simulink model "rfdctxrx"  (R2025a)
settings: Solver=VariableStepAuto  StartTime=0.0  StopTime=10.0  RelTol=1e-3
libraries: hdlBasic x265, casper_library_misc x2, xps_library x1, vmcUtilities x1
(part 5 of 7)

== system rfdctxrx/tx_enable ==
  sim_1 : Inport
  convert1_1 : DataTypeConversion  OutDataTypeStr=fixdt('ufix1_En0')  SaturateOnIntegerOverflow=off  RndMeth=Floor  LockScale=on
  convert2_1 : DataTypeConversion  OutDataTypeStr=fixdt('ufix1_En0')  ConvertRealWorld=Stored Integer (SI)  SaturateOnIntegerOverflow=off  RndMeth=Floor  LockScale=on
  gain_1 : Gain  OutDataTypeStr=fixdt('ufix32_En0')
  io_delay : hdlBasic/Delay  rst=off  en=off  latency=0  reg_retiming=on  XmcBlockStatus=0  maskContainerNames=group1  block_type=delay  block_config=sysgen:Delay_config
  rfdctxrx_tx_enable_user_data_out : hdlBasic/Gateway In  gui_display_data_type=Fixed-point  arith_type=Unsigned  n_bits=32  bin_pt=0  preci_type=Single  exp_width=8  frac_width=24  rows=1  columns=1  quantization="Round  (unbiased: +/- Inf)"  overflow=Saturate  period=1  UseAsADC=off  ADCChannel='1'  interface=None  automatic_assignment=on  address_offset=hex2dec('00')  intf_name=''  intf_description=''  default_value=0  timing_constraint=None  locs_specified=off  LOCs={}  io_standard={}  inherit_from_input=off  hdl_port=on  XmcBlockStatus=0  maskContainerNames=group4  block_type=gatewayin  block_config=sysgen:gateway_in_config  block_width_w=590  block_height_w=620  block_width=640  block_height=850
  slice_reg : hdlBasic/Slice  nbits=1  boolean_output=on  mode=Lower Bit Location + Width  bit1=0  base1=MSB of Input  bit0=0  base0=LSB of Input  XmcBlockStatus=0  maskContainerNames=group1  block_type=slice  block_config=sysgen:Slice_config
  in_reg : Outport
  wires:
  rfdctxrx_tx_enable_user_data_out/1 -> io_delay/1
  sim_1/1 -> convert1_1/1
  convert1_1/1 -> convert2_1/1
  convert2_1/1 -> gain_1/1
  gain_1/1 -> rfdctxrx_tx_enable_user_data_out/1
  io_delay/1 -> slice_reg/1
  slice_reg/1 -> in_reg/1

== system rfdctxrx/tx_len ==
  out_reg : Inport
  assert_reg : hdlBasic/Assert  assert_type=on  type_source=Explicitly  gui_display_data_type=Fixed-point  arith_type=Unsigned  n_bits=13  bin_pt=0  preci_type=Single  exp_width=8  frac_width=24  assert_rate=off  rate_source=Explicitly  period=1  output_port=on  XmcBlockStatus=0  maskContainerNames=group1  block_type=assert  block_config=sysgen:assert_config  block_width=609  block_height=900
  cast_gw : hdlBasic/Convert  gui_display_data_type=Fixed-point  arith_type=Unsigned  n_bits=32  bin_pt=0  float_type=Single  exp_bits=8  fraction_bits=24  quantization=Truncate  overflow=Wrap  en=off  latency=1  pipeline=off  XmcBlockStatus=0  maskContainerNames=group2  block_type=convert  block_config=sysgen:Convert_config  block_width=595  block_height=885
  io_delay : hdlBasic/Delay  rst=off  en=off  latency=0  reg_retiming=on  XmcBlockStatus=0  maskContainerNames=group1  block_type=delay  block_config=sysgen:Delay_config
  reint1 : hdlBasic/Reinterpret  force_arith_type=on  arith_type=Unsigned  force_bin_pt=on  bin_pt=0  XmcBlockStatus=0  maskContainerNames=group1  block_type=reinterpret  block_config=sysgen:Reinterpret_config
  rfdctxrx_tx_len_user_data_in : hdlBasic/Gateway Out  inherit_from_input=off  bool_to_boolean=off  hdl_port=on  rows=1  columns=1  UseAsDAC=off  DACChannel='1'  interface=None  automatic_assignment=on  address_offset=hex2dec('00')  intf_name=''  intf_description=''  timing_constraint=None  locs_specified=off  LOCs={}  io_standard={}  XmcBlockStatus=0  maskContainerNames=group4  block_type=gatewayout  block_config=sysgen:gateway_out_config  block_width_w=590  block_height_w=620  block_width=620  block_height=750
  sim_out : Terminator
  sim_out_reg_gw : hdlBasic/Gateway Out  inherit_from_input=off  bool_to_boolean=off  hdl_port=off  rows=1  columns=1  UseAsDAC=off  DACChannel='1'  interface=None  automatic_assignment=on  address_offset=hex2dec('00')  intf_name=''  intf_description=''  timing_constraint=None  locs_specified=off  LOCs={}  io_standard={}  XmcBlockStatus=0  maskContainerNames=group4  block_type=gatewayout  block_config=sysgen:gateway_out_config  block_width_w=590  block_height_w=620  block_width=620  block_height=750
  sim_out_reg_sim_delay : hdlBasic/Delay  rst=off  en=off  latency=1  reg_retiming=on  XmcBlockStatus=0  maskContainerNames=group1  block_type=delay  block_config=sysgen:Delay_config
  sim_out_reg : Outport  VectorParamsAs1DForOutWhenUnconnected=off
  wires:
  sim_out_reg_sim_delay/1 -> sim_out_reg_gw/1
  sim_out_reg_gw/1 -> sim_out_reg/1
  io_delay/1 -> cast_gw/1
  cast_gw/1 -> rfdctxrx_tx_len_user_data_in/1
  rfdctxrx_tx_len_user_data_in/1 -> sim_out/1
  out_reg/1 -> sim_out_reg_sim_delay/1, assert_reg/1
  assert_reg/1 -> reint1/1
  reint1/1 -> io_delay/1

== system rfdctxrx/bitfield_snapshot/buscreate ==
  in1 : Inport
  in2 : Inport  Port=2
  concatenate : hdlBasic/Concat  num_inputs=2  XmcBlockStatus=1  maskContainerNames=group1  block_type=concat  block_config=sysgen:Concat_config
  reinterpret1 : hdlBasic/Reinterpret  force_arith_type=on  arith_type=Unsigned  force_bin_pt=on  bin_pt=0  XmcBlockStatus=1  maskContainerNames=group1  block_type=reinterpret  block_config=sysgen:Reinterpret_config
  reinterpret2 : hdlBasic/Reinterpret  force_arith_type=on  arith_type=Unsigned  force_bin_pt=on  bin_pt=0  XmcBlockStatus=1  maskContainerNames=group1  block_type=reinterpret  block_config=sysgen:Reinterpret_config
  bus_out : Outport  VectorParamsAs1DForOutWhenUnconnected=off
  wires:
  concatenate/1 -> bus_out/1
  in1/1 -> reinterpret1/1
  reinterpret1/1 -> concatenate/1
  in2/1 -> reinterpret2/1
  reinterpret2/1 -> concatenate/2

== system rfdctxrx/bitfield_snapshot/io_delay ==
  d : Inport
  Register0 : hdlBasic/Register  init=0  rst=off  en=off  XmcBlockStatus=1  maskContainerNames=tabcontainer1  block_type=register  block_config=sysgen:Register_config
  Register1 : hdlBasic/Register  init=0  rst=off  en=off  XmcBlockStatus=1  maskContainerNames=tabcontainer1  block_type=register  block_config=sysgen:Register_config
  q : Outport  VectorParamsAs1DForOutWhenUnconnected=off
  wires:
  Register1/1 -> q/1
  d/1 -> Register0/1
  Register0/1 -> Register1/1

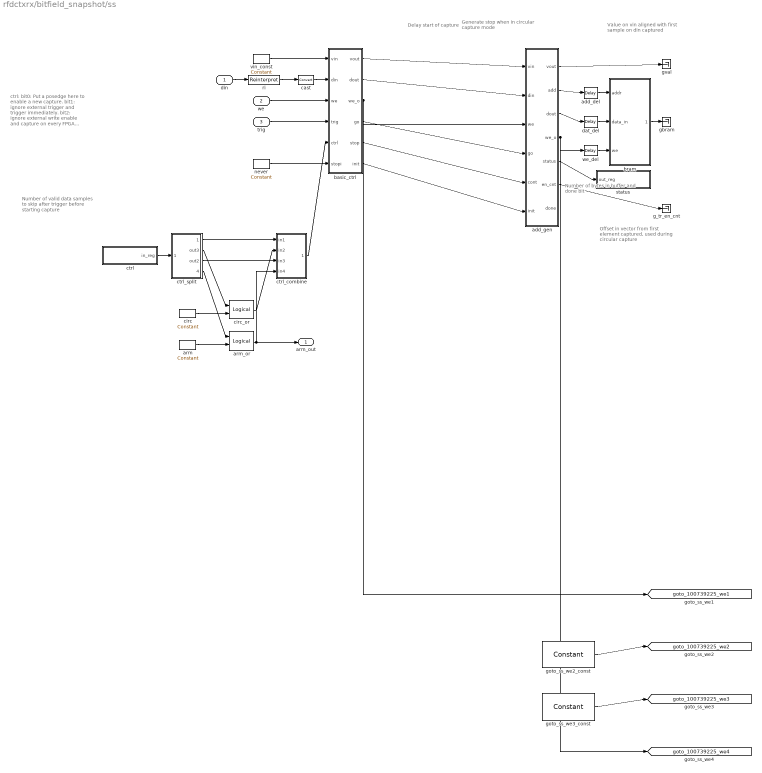
== system rfdctxrx/bitfield_snapshot/ss ==
  note: Generate stop
      | when in circular
      | capture mode
  note: Delay start
      | of capture
  note: ctrl:
      | bit0: Put a posedge here
      |         to enable a new capture.
      | bit1: ignore external trigger
      |         and trigger immediately.
      | bit2: ignore external write
      |         enable and capture on
      |         every FPGA clock.
      | bit3: continuously capture
      |         data until we get an
      |         external stop command.
  note: Offset in vector
      | from first element
      | captured, used
      | during circular capture
  note: Number of
      | bytes in
      | buffer and
      | done bit
  note: Number of valid
      | data samples to
      | skip after trigger
      | before starting
      | capture
  note: Value on vin
      | aligned with
      | first sample on
      | din captured
  din : Inport
  we : Inport  Port=2
  trig : Inport  Port=3
  add_del : hdlBasic/Delay  rst=off  en=off  latency=1  reg_retiming=off  XmcBlockStatus=1  maskContainerNames=group1  block_type=delay  block_config=sysgen:Delay_config
  add_gen : Subsystem  AncestorBlock=casper_library_scopes/snapshot/add_gen  mask{counter_size=14+4+1, increment=16, nsamples=14, burst_size=0, use_dsp48=on}
      mask prompts: counter_size "Address counter size (2^?)"; increment "Address counter increment"; nsamples "Number of samples (2^?)"; burst_size "Burst size (2^?)"; use_dsp48 "dsp48 counter/s"
      mask init:
      | set_param(gcb,'LinkStatus','inactive');
      | if strcmp(use_dsp48,'on'),
      |     set_param([gcb,'/add_gen'],'implementation','DSP48');
      | else
      |     set_param([gcb,'/add_gen'],'implementation','Fabric');
      | end
  arm : hdlBasic/Constant  const=0  gui_display_data_type=Boolean  arith_type=Boolean  n_bits=16  bin_pt=14  preci_type=Single  exp_width=8  frac_width=24  explicit_period=on  period=1  XmcBlockStatus=1  maskContainerNames=tabcontainer1  block_type=constant  block_config=sysgen:Constant_config
  arm_or : hdlBasic/Logical  logical_function=OR  inputs=2  en=off  latency=0  precision=Full  arith_type=Unsigned  n_bits=16  bin_pt=0  align_bp=on  overflow=[]  quantization=[]  XmcBlockStatus=1  maskContainerNames=tabcontainer1  block_type=logical  block_config=sysgen:Logical_config
  basic_ctrl : Subsystem  AncestorBlock=casper_library_scopes/snapshot/basic_ctrl  mask{dram=off, data_width=128}
      mask prompts: data_width "data width"
      mask init:
      | set_param(gcb,'LinkStatus','inactive');
      | set_param([gcb,'/dram_munge'], 'dram', dram);
  bram : Subsystem  Tag=xps:bram  AncestorBlock=xps_library/Memory/shared_bram  mask{arith_type=Unsigned, addr_width=14, data_width=128, reg_prim_output=off, reg_core_output=off, optimization=Minimum_Area, data_bin_pt=0, init_vals=[0:2^14-1], sample_rate=1}
      mask prompts: arith_type "Output Data Type"; addr_width "Address width"; data_width "Data Width"; reg_prim_output "Register Primitive Output"; reg_core_output "Register Core Output"; data_bin_pt "Data Binary Point"; init_vals "Initial values (simulation only)"; sample_rate "Sample rate"
      mask init:
      | shared_bram_mask;
      mask TypeOptions arith_type: Unsigned | Signed  (2's comp)
      mask TypeOptions data_width: 8 | 16 | 32 | 64 | 128
      mask TypeOptions optimization: Minimum_Area | Low_Power
  cast : hdlBasic/Convert  gui_display_data_type=Fixed-point  arith_type=Unsigned  n_bits=128  bin_pt=0  float_type=Single  exp_bits=8  fraction_bits=24  quantization=Truncate  overflow=Wrap  en=off  latency=0  pipeline=off  XmcBlockStatus=1  maskContainerNames=group2  block_type=convert  block_config=sysgen:Convert_config  block_width=595  block_height=885
  circ : hdlBasic/Constant  const=0  gui_display_data_type=Boolean  arith_type=Boolean  n_bits=16  bin_pt=14  preci_type=Single  exp_width=8  frac_width=24  explicit_period=on  period=1  XmcBlockStatus=1  maskContainerNames=tabcontainer1  block_type=constant  block_config=sysgen:Constant_config
  circ_or : hdlBasic/Logical  logical_function=OR  inputs=2  en=off  latency=0  precision=Full  arith_type=Unsigned  n_bits=16  bin_pt=0  align_bp=on  overflow=[]  quantization=[]  XmcBlockStatus=1  maskContainerNames=tabcontainer1  block_type=logical  block_config=sysgen:Logical_config
  ctrl : Subsystem  Tag=xps:sw_reg  AncestorBlock=xps_library/Memory/software_register  mask(swreg){io_dir=From Processor, io_delay=0, init_val=0, sample_period=1, names=reg, bitwidths=32, bin_pts=0, arith_types=0, sim_port=off, show_format=on}
      mask prompts: io_dir "I/O direction"; io_delay "I/O delay"; init_val "Initial Value"; sample_period "Sample period"; names "Bitfield names [msb...lsb]"; bitwidths "Bitfield widths"; bin_pts "Bitfield binary pts"; arith_types "Bitfield types, ufix=0, fix=1, bool=2"; sim_port "Provide sim input/output?"; show_format "Print format string?"
      mask help: A 32-bit software-accessible register. Can be divided into bitfields of varying widths and types using the fields in the block mask.
      mask init:
      | swreg_init(gcb)
      settings: AttributesFormatString=1input:uf32.0 = 32 bits
      mask TypeOptions io_dir: To Processor | From Processor
      mask Callback io_dir:
      | mask_enables = get_param(gcb, 'MaskEnables');
      | mask_names = get_param(gcb, 'MaskNames');
      | if strcmp(get_param(gcb, 'io_dir'), 'To Processor'),
      |     mask_enables{ismember(mask_names, 'sample_period')} = 'off';
      | else
      |     mask_enables{ismember(mask_names, 'sample_period')} = 'on';
      | end
      | set_param(gcb, 'MaskEnables', mask_enables);
      mask DialogControl ParameterTabVar0 Prompt: Setup
  ctrl_combine : Subsystem  AncestorBlock=casper_library_flow_control/bus_create  mask(bus_create){inputNum=4}
      mask prompts: inputNum "Number of inputs:"
      mask init:
      | bus_create_init(gcb,...
      |     'inputNum', inputNum);
  ctrl_split : Subsystem  AncestorBlock=casper_library_flow_control/bus_expand  mask(bus_expand){mode=divisions of arbitrary size, outputNum=1, outputWidth=[28 1 2 1], outputBinaryPt=0, outputArithmeticType=[0 2 0 2], show_format=on, outputToWorkspace=off, variablePrefix=out, outputToModelAsWell=on}
      mask prompts: outputNum "Number of outputs:"; outputWidth "Output width [msb ... lsb]:"; outputBinaryPt "Output binary point position [msb ... lsb]:"; outputArithmeticType "Output arithmetic type (ufix=0, fix=1, bool=2) [msb ... lsb]:"; show_format "Print format string?"; outputToWorkspace "Output to workspace?"; variablePrefix "Variable name prefix:"; outputToModelAsWell "Output to model as well?"
      mask help:
      | Expands a 'bus' made using a bus_create or Xilinx
      | concat block.
      | The input will be divided into the specified number
      | of outputs with the specified arithmetic types.
      | Divisions are made from most significant bit.
      mask init: same as rfdctxrx/munge/split
      settings: AttributesFormatString=4 outputs: uf28.0,b,uf2.0,b,
      mask TypeOptions mode: divisions of equal size | divisions of arbitrary size
      mask Callback mode: bus_expand_callback();
      mask Callback outputWidth: bus_expand_callback();
      mask Callback outputToWorkspace: bus_expand_callback();
  dat_del : hdlBasic/Delay  rst=off  en=off  latency=1  reg_retiming=off  XmcBlockStatus=1  maskContainerNames=group1  block_type=delay  block_config=sysgen:Delay_config
  g_tr_en_cnt : Terminator
  gbram : Terminator
  goto_ss_we2_const : hdlBasic/Constant  const=0  gui_display_data_type=Boolean  arith_type=Boolean  n_bits=16  bin_pt=14  preci_type=Single  exp_width=8  frac_width=24  explicit_period=on  period=1  XmcBlockStatus=1  maskContainerNames=tabcontainer1  block_type=constant  block_config=sysgen:Constant_config
  goto_ss_we3_const : hdlBasic/Constant  const=0  gui_display_data_type=Boolean  arith_type=Boolean  n_bits=16  bin_pt=14  preci_type=Single  exp_width=8  frac_width=24  explicit_period=on  period=1  XmcBlockStatus=1  maskContainerNames=tabcontainer1  block_type=constant  block_config=sysgen:Constant_config
  gval : Terminator
  never : hdlBasic/Constant  const=0  gui_display_data_type=Boolean  arith_type=Boolean  n_bits=16  bin_pt=14  preci_type=Single  exp_width=8  frac_width=24  explicit_period=on  period=1  XmcBlockStatus=1  maskContainerNames=tabcontainer1  block_type=constant  block_config=sysgen:Constant_config
  ri : hdlBasic/Reinterpret  force_arith_type=on  arith_type=Unsigned  force_bin_pt=on  bin_pt=0  XmcBlockStatus=1  maskContainerNames=group1  block_type=reinterpret  block_config=sysgen:Reinterpret_config
  status : Subsystem  Tag=xps:sw_reg  AncestorBlock=xps_library/Memory/software_register  mask(swreg){io_dir=To Processor, io_delay=0, init_val=0, sample_period=1, names=reg, bitwidths=32, bin_pts=0, arith_types=0, sim_port=off, show_format=on}
      mask prompts: io_dir "I/O direction"; io_delay "I/O delay"; init_val "Initial Value"; sample_period "Sample period"; names "Bitfield names [msb...lsb]"; bitwidths "Bitfield widths"; bin_pts "Bitfield binary pts"; arith_types "Bitfield types, ufix=0, fix=1, bool=2"; sim_port "Provide sim input/output?"; show_format "Print format string?"
      mask help: A 32-bit software-accessible register. Can be divided into bitfields of varying widths and types using the fields in the block mask.
      mask init:
      | swreg_init(gcb)
      settings: AttributesFormatString=1output:uf32.0 = 32 bits
      mask TypeOptions io_dir: To Processor | From Processor
      mask Callback io_dir:
      | mask_enables = get_param(gcb, 'MaskEnables');
      | mask_names = get_param(gcb, 'MaskNames');
      | if strcmp(get_param(gcb, 'io_dir'), 'To Processor'),
      |     mask_enables{ismember(mask_names, 'sample_period')} = 'off';
      | else
      |     mask_enables{ismember(mask_names, 'sample_period')} = 'on';
      | end
      | set_param(gcb, 'MaskEnables', mask_enables);
      mask DialogControl ParameterTabVar0 Prompt: Setup
  vin_const : hdlBasic/Constant  const=0  gui_display_data_type=Boolean  arith_type=Boolean  n_bits=16  bin_pt=14  preci_type=Single  exp_width=8  frac_width=24  explicit_period=on  period=1  XmcBlockStatus=1  maskContainerNames=tabcontainer1  block_type=constant  block_config=sysgen:Constant_config
  we_del : hdlBasic/Delay  rst=off  en=off  latency=1  reg_retiming=off  XmcBlockStatus=1  maskContainerNames=group1  block_type=delay  block_config=sysgen:Delay_config
  arm_out : Outport  VectorParamsAs1DForOutWhenUnconnected=off
  tag scope: goto_100739225_we1=global, goto_100739225_we2=global, goto_100739225_we3=global, goto_100739225_we4=global
  wires:
  din/1 -> ri/1
  ri/1 -> cast/1
  cast/1 -> basic_ctrl/2(din)
  we/1 -> basic_ctrl/3(we)
  trig/1 -> basic_ctrl/4(trig)
  ctrl_combine/1(bus_out) -> basic_ctrl/5(ctrl)
  never/1 -> basic_ctrl/6(stopi)
  arm/1 -> arm_or/2
  arm_or/1 -> arm_out/1, ctrl_combine/4(in4)
  circ/1 -> circ_or/2
  ctrl/1(in_reg) -> ctrl_split/1(bus_in)
  ctrl_split/1(msb_out4) -> ctrl_combine/1(in1)
  ctrl_split/2(out3) -> circ_or/1
  ctrl_split/3(out2) -> ctrl_combine/3(in3)
  ctrl_split/4(lsb_out1) -> arm_or/1
  circ_or/1 -> ctrl_combine/2(in2)
  basic_ctrl/1(vout) -> add_gen/1(vin)
  basic_ctrl/2(dout) -> add_gen/2(din)
  basic_ctrl/3(we_o) -> add_gen/3(we), [goto_100739225_we1]
  basic_ctrl/4(go) -> add_gen/4(go)
  basic_ctrl/5(stop) -> add_gen/5(cont)
  basic_ctrl/6(init) -> add_gen/6(init)
  add_gen/5(status) -> status/1(out_reg)
  vin_const/1 -> basic_ctrl/1(vin)
  add_gen/1(vout) -> gval/1
  add_gen/6(en_cnt) -> g_tr_en_cnt/1
  add_gen/2(add) -> add_del/1
  add_gen/3(dout) -> dat_del/1
  add_gen/4(we_o) -> we_del/1, [goto_100739225_we4]
  add_del/1 -> bram/1(addr)
  dat_del/1 -> bram/2(data_in)
  we_del/1 -> bram/3(we)
  bram/1(data_out) -> gbram/1
  goto_ss_we2_const/1 -> [goto_100739225_we2]
  goto_ss_we3_const/1 -> [goto_100739225_we3]

== system rfdctxrx/bitfield_snapshot/trig_delay ==
  d : Inport
  Register0 : hdlBasic/Register  init=0  rst=off  en=off  XmcBlockStatus=1  maskContainerNames=tabcontainer1  block_type=register  block_config=sysgen:Register_config
  Register1 : hdlBasic/Register  init=0  rst=off  en=off  XmcBlockStatus=1  maskContainerNames=tabcontainer1  block_type=register  block_config=sysgen:Register_config
  q : Outport  VectorParamsAs1DForOutWhenUnconnected=off
  wires:
  Register1/1 -> q/1
  d/1 -> Register0/1
  Register0/1 -> Register1/1

== system rfdctxrx/bitfield_snapshot/we_delay ==
  d : Inport
  Register0 : hdlBasic/Register  init=0  rst=off  en=off  XmcBlockStatus=1  maskContainerNames=tabcontainer1  block_type=register  block_config=sysgen:Register_config
  Register1 : hdlBasic/Register  init=0  rst=off  en=off  XmcBlockStatus=1  maskContainerNames=tabcontainer1  block_type=register  block_config=sysgen:Register_config
  q : Outport  VectorParamsAs1DForOutWhenUnconnected=off
  wires:
  Register1/1 -> q/1
  d/1 -> Register0/1
  Register0/1 -> Register1/1

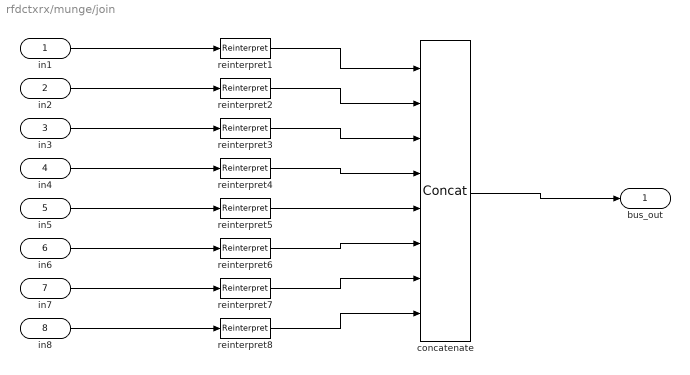
== system rfdctxrx/munge/join ==
  in1 : Inport
  in2 : Inport  Port=2
  in3 : Inport  Port=3
  in4 : Inport  Port=4
  in5 : Inport  Port=5
  in6 : Inport  Port=6
  in7 : Inport  Port=7
  in8 : Inport  Port=8
  concatenate : hdlBasic/Concat  num_inputs=8  XmcBlockStatus=1  maskContainerNames=group1  block_type=concat  block_config=sysgen:Concat_config
  reinterpret{1..8} (8 alike) : hdlBasic/Reinterpret  force_arith_type=on  arith_type=Unsigned  force_bin_pt=on  bin_pt=0  XmcBlockStatus=1  maskContainerNames=group1  block_type=reinterpret  block_config=sysgen:Reinterpret_config
  bus_out : Outport  VectorParamsAs1DForOutWhenUnconnected=off
  wires:
  concatenate/1 -> bus_out/1
  in1/1 -> reinterpret1/1
  reinterpret1/1 -> concatenate/1
  in2/1 -> reinterpret2/1
  reinterpret2/1 -> concatenate/2
  in3/1 -> reinterpret3/1
  reinterpret3/1 -> concatenate/3
  in4/1 -> reinterpret4/1
  reinterpret4/1 -> concatenate/4
  in5/1 -> reinterpret5/1
  reinterpret5/1 -> concatenate/5
  in6/1 -> reinterpret6/1
  reinterpret6/1 -> concatenate/6
  in7/1 -> reinterpret7/1
  reinterpret7/1 -> concatenate/7
  in8/1 -> reinterpret8/1
  reinterpret8/1 -> concatenate/8

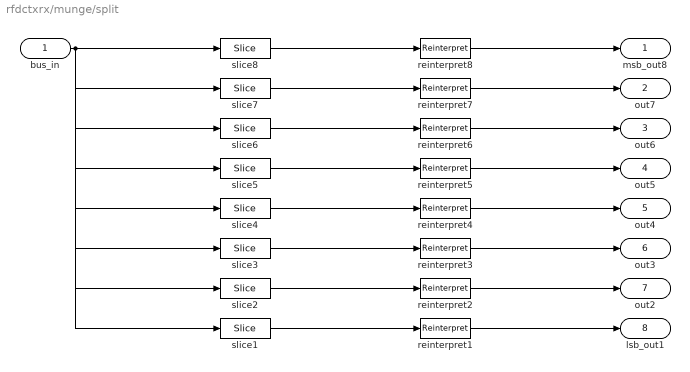
== system rfdctxrx/munge/split ==
  bus_in : Inport
  reinterpret{1..8} (8 alike) : hdlBasic/Reinterpret  force_arith_type=on  arith_type=Unsigned  force_bin_pt=on  bin_pt=0  XmcBlockStatus=1  maskContainerNames=group1  block_type=reinterpret  block_config=sysgen:Reinterpret_config
  slice1 : hdlBasic/Slice  nbits=16  boolean_output=off  mode=Upper Bit Location + Width  bit1=-112  base1=MSB of Input  bit0=0  base0=LSB of Input  XmcBlockStatus=1  maskContainerNames=group1  block_type=slice  block_config=sysgen:Slice_config
  slice2 : hdlBasic/Slice  nbits=16  boolean_output=off  mode=Upper Bit Location + Width  bit1=-96  base1=MSB of Input  bit0=0  base0=LSB of Input  XmcBlockStatus=1  maskContainerNames=group1  block_type=slice  block_config=sysgen:Slice_config
  slice3 : hdlBasic/Slice  nbits=16  boolean_output=off  mode=Upper Bit Location + Width  bit1=-80  base1=MSB of Input  bit0=0  base0=LSB of Input  XmcBlockStatus=1  maskContainerNames=group1  block_type=slice  block_config=sysgen:Slice_config
  slice4 : hdlBasic/Slice  nbits=16  boolean_output=off  mode=Upper Bit Location + Width  bit1=-64  base1=MSB of Input  bit0=0  base0=LSB of Input  XmcBlockStatus=1  maskContainerNames=group1  block_type=slice  block_config=sysgen:Slice_config
  slice5 : hdlBasic/Slice  nbits=16  boolean_output=off  mode=Upper Bit Location + Width  bit1=-48  base1=MSB of Input  bit0=0  base0=LSB of Input  XmcBlockStatus=1  maskContainerNames=group1  block_type=slice  block_config=sysgen:Slice_config
  slice6 : hdlBasic/Slice  nbits=16  boolean_output=off  mode=Upper Bit Location + Width  bit1=-32  base1=MSB of Input  bit0=0  base0=LSB of Input  XmcBlockStatus=1  maskContainerNames=group1  block_type=slice  block_config=sysgen:Slice_config
  slice7 : hdlBasic/Slice  nbits=16  boolean_output=off  mode=Upper Bit Location + Width  bit1=-16  base1=MSB of Input  bit0=0  base0=LSB of Input  XmcBlockStatus=1  maskContainerNames=group1  block_type=slice  block_config=sysgen:Slice_config
  slice8 : hdlBasic/Slice  nbits=16  boolean_output=off  mode=Upper Bit Location + Width  bit1=0  base1=MSB of Input  bit0=0  base0=LSB of Input  XmcBlockStatus=1  maskContainerNames=group1  block_type=slice  block_config=sysgen:Slice_config
  msb_out8 : Outport
  out7 : Outport  Port=2
  out6 : Outport  Port=3
  out5 : Outport  Port=4
  out4 : Outport  Port=5
  out3 : Outport  Port=6
  out2 : Outport  Port=7
  lsb_out1 : Outport  Port=8  VectorParamsAs1DForOutWhenUnconnected=off
  wires:
  bus_in/1 -> slice8/1, slice7/1, slice6/1, slice5/1, slice4/1, slice3/1, slice2/1, slice1/1
  slice8/1 -> reinterpret8/1
  reinterpret8/1 -> msb_out8/1
  slice7/1 -> reinterpret7/1
  reinterpret7/1 -> out7/1
  slice6/1 -> reinterpret6/1
  reinterpret6/1 -> out6/1
  slice5/1 -> reinterpret5/1
  reinterpret5/1 -> out5/1
  slice4/1 -> reinterpret4/1
  reinterpret4/1 -> out4/1
  slice3/1 -> reinterpret3/1
  reinterpret3/1 -> out3/1
  slice2/1 -> reinterpret2/1
  reinterpret2/1 -> out2/1
  slice1/1 -> reinterpret1/1
  reinterpret1/1 -> lsb_out1/1

== system rfdctxrx/tx_bram/calc_add ==
  note: Use behavioural HDL
      | so that gets optimised
      | to minimum logic
  note: If reading/writing words
      | smaller than 32 bits,
      | change address so
      | that addressing is
      | big endian instead of
      | little, otherwise
      | pass through
  in : Inport
  add_sub : hdlBasic/AddSub  mode=Subtraction  use_carryin=off  use_carryout=off  en=off  latency=0  precision=User Defined  arith_type=Unsigned  n_bits=max(1, log2(32/data_width))  bin_pt=0  quantization=Truncate  overflow=Wrap  use_behavioral_HDL=on  hw_selection=Fabric  pipelined=off  XmcBlockStatus=1  maskContainerNames=tabcontainer1  block_type=addsub  block_config=sysgen:Addsub_config
  concat : hdlBasic/Concat  num_inputs=2  XmcBlockStatus=1  maskContainerNames=group1  block_type=concat  block_config=sysgen:Concat_config
  const : hdlBasic/Constant  const=max(0, 32/data_width-1)  gui_display_data_type=Fixed-point  arith_type=Unsigned  n_bits=max(1, log2(32/data_width))  bin_pt=0  preci_type=Single  exp_width=8  frac_width=24  explicit_period=on  period=sample_rate  XmcBlockStatus=1  maskContainerNames=tabcontainer1  block_type=constant  block_config=sysgen:Constant_config
  convert_addr : hdlBasic/Convert  gui_display_data_type=Fixed-point  arith_type=Unsigned  n_bits=addr_width  bin_pt=0  float_type=Single  exp_bits=8  fraction_bits=24  quantization=Truncate  overflow=Wrap  en=off  latency=0  pipeline=off  XmcBlockStatus=1  maskContainerNames=group2  block_type=convert  block_config=sysgen:Convert_config  block_width=595  block_height=885
  lsw : hdlBasic/Slice  nbits=max(1, log2(32/data_width))  boolean_output=off  mode=Lower Bit Location + Width  bit1=0  base1=MSB of Input  bit0=0  base0=LSB of Input  XmcBlockStatus=1  maskContainerNames=group1  block_type=slice  block_config=sysgen:Slice_config
  manipulate : hdlBasic/Constant  const=min(1, floor(32/data_width) - 1)  gui_display_data_type=Fixed-point  arith_type=Unsigned  n_bits=1  bin_pt=0  preci_type=Single  exp_width=8  frac_width=24  explicit_period=on  period=sample_rate  XmcBlockStatus=1  maskContainerNames=tabcontainer1  block_type=constant  block_config=sysgen:Constant_config
  msw : hdlBasic/Slice  nbits=addr_width - max(1, log2(32/data_width))  boolean_output=off  mode=Upper Bit Location + Width  bit1=0  base1=MSB of Input  bit0=0  base0=LSB of Input  XmcBlockStatus=1  maskContainerNames=group1  block_type=slice  block_config=sysgen:Slice_config
  mux : hdlBasic/Mux  inputs=2  en=off  latency=0  precision=Full  arith_type=Unsigned  n_bits=16  bin_pt=14  quantization=Truncate  overflow=Wrap  XmcBlockStatus=1  maskContainerNames=tabcontainer1  block_type=mux  block_config=sysgen:Mux_config
  out : Outport  VectorParamsAs1DForOutWhenUnconnected=off
  wires:
  convert_addr/1 -> mux/2, msw/1, lsw/1
  const/1 -> add_sub/1
  lsw/1 -> add_sub/2
  mux/1 -> out/1
  manipulate/1 -> mux/1
  concat/1 -> mux/3
  msw/1 -> concat/1
  add_sub/1 -> concat/2
  in/1 -> convert_addr/1

== system rfdctxrx/tx_bram/munge_in ==
  din : Inport
  join : Subsystem  AncestorBlock=casper_library_flow_control/bus_create  mask(bus_create){inputNum=4}
      mask prompts: inputNum "Number of inputs:"
      mask init:
      | bus_create_init(gcb,...
      |     'inputNum', inputNum);
  reinterpret : hdlBasic/Reinterpret  force_arith_type=on  arith_type=Unsigned  force_bin_pt=on  bin_pt=0  XmcBlockStatus=1  maskContainerNames=group1  block_type=reinterpret  block_config=sysgen:Reinterpret_config
  reinterpret_out : hdlBasic/Reinterpret  force_arith_type=on  arith_type=Unsigned  force_bin_pt=on  bin_pt=0  XmcBlockStatus=1  maskContainerNames=group1  block_type=reinterpret  block_config=sysgen:Reinterpret_config
  split : Subsystem  AncestorBlock=casper_library_flow_control/bus_expand  mask(bus_expand){mode=divisions of arbitrary size, outputNum=4, outputWidth=[32 32 32 32], outputBinaryPt=[0 0 0 0], outputArithmeticType=[0 0 0 0], show_format=off, outputToWorkspace=off, variablePrefix=out, outputToModelAsWell=on}
      mask prompts: outputNum "Number of outputs:"; outputWidth "Output width:"; outputBinaryPt "Output binary point position:"; outputArithmeticType "Output arithmetic type (ufix=0, fix=1, bool=2):"; show_format "Print format string?"; outputToWorkspace "Output to workspace?"; variablePrefix "Variable name prefix:"; outputToModelAsWell "Output to model as well?"
      mask help:
      | Expands a 'bus' made using a bus_create or Xilinx
      | concat block.
      | The input will be divided into the specified number
      | of outputs with the specified arithmetic types.
      | Divisions are made from most significant bit.
      mask init: same as rfdctxrx/munge/split
      settings: AttributesFormatString=4 outputs
      mask TypeOptions mode: divisions of equal size | divisions of arbitrary size
      mask Callback mode: %bus_expand_callback();
      mask Callback outputWidth: %bus_expand_callback();
      mask Callback outputToWorkspace: %bus_expand_callback();
  dout : Outport  VectorParamsAs1DForOutWhenUnconnected=off
  wires:
  reinterpret_out/1 -> dout/1
  din/1 -> reinterpret/1
  reinterpret/1 -> split/1(bus_in)
  join/1(bus_out) -> reinterpret_out/1
  split/4(lsb_out1) -> join/1(in1)
  split/3(out2) -> join/2(in2)
  split/2(out3) -> join/3(in3)
  split/1(msb_out4) -> join/4(in4)

== system rfdctxrx/tx_bram/munge_out ==
  din : Inport
  join : Subsystem  AncestorBlock=casper_library_flow_control/bus_create  mask(bus_create){inputNum=4}
      mask prompts: inputNum "Number of inputs:"
      mask init:
      | bus_create_init(gcb,...
      |     'inputNum', inputNum);
  reinterpret : hdlBasic/Reinterpret  force_arith_type=on  arith_type=Unsigned  force_bin_pt=on  bin_pt=0  XmcBlockStatus=1  maskContainerNames=group1  block_type=reinterpret  block_config=sysgen:Reinterpret_config
  reinterpret_out : hdlBasic/Reinterpret  force_arith_type=on  arith_type=Unsigned  force_bin_pt=on  bin_pt=0  XmcBlockStatus=1  maskContainerNames=group1  block_type=reinterpret  block_config=sysgen:Reinterpret_config
  split : Subsystem  AncestorBlock=casper_library_flow_control/bus_expand  mask(bus_expand){mode=divisions of arbitrary size, outputNum=4, outputWidth=[32 32 32 32], outputBinaryPt=[0 0 0 0], outputArithmeticType=[0 0 0 0], show_format=off, outputToWorkspace=off, variablePrefix=out, outputToModelAsWell=on}
      mask prompts: outputNum "Number of outputs:"; outputWidth "Output width:"; outputBinaryPt "Output binary point position:"; outputArithmeticType "Output arithmetic type (ufix=0, fix=1, bool=2):"; show_format "Print format string?"; outputToWorkspace "Output to workspace?"; variablePrefix "Variable name prefix:"; outputToModelAsWell "Output to model as well?"
      mask help:
      | Expands a 'bus' made using a bus_create or Xilinx
      | concat block.
      | The input will be divided into the specified number
      | of outputs with the specified arithmetic types.
      | Divisions are made from most significant bit.
      mask init: same as rfdctxrx/munge/split
      settings: AttributesFormatString=4 outputs
      mask TypeOptions mode: divisions of equal size | divisions of arbitrary size
      mask Callback mode: %bus_expand_callback();
      mask Callback outputWidth: %bus_expand_callback();
      mask Callback outputToWorkspace: %bus_expand_callback();
  dout : Outport  VectorParamsAs1DForOutWhenUnconnected=off
  wires:
  reinterpret_out/1 -> dout/1
  din/1 -> reinterpret/1
  reinterpret/1 -> split/1(bus_in)
  join/1(bus_out) -> reinterpret_out/1
  split/4(lsb_out1) -> join/1(in1)
  split/3(out2) -> join/2(in2)
  split/2(out3) -> join/3(in3)
  split/1(msb_out4) -> join/4(in4)

== system rfdctxrx/tx_bram/sim_mem ==
  addr : Inport
  data : Inport  Port=2
  we : Inport  Port=3
  Data Type Conversion : DataTypeConversion  OutDataTypeStr=single  SaturateOnIntegerOverflow=off  RndMeth=Floor
  Data Type Conversion1 : DataTypeConversion  OutDataTypeStr=double  SaturateOnIntegerOverflow=off  RndMeth=Floor
  Data Type Conversion2 : DataTypeConversion  OutDataTypeStr=boolean  SaturateOnIntegerOverflow=off  RndMeth=Floor
  sfunc : M-S-Function  FunctionName=shared_bram_sim_sfunc  Parameters=depth_bits, latency, init_vals  mask{depth_bits=addr_width, latency=csp_latency, init_vals=init_vals}
      mask prompts: depth_bits "Depth (2^?):"; latency "Latency (>=1):"; init_vals "Initial values:"
      mask Callback latency:
      | latency = str2double(get_param(gcb, 'latency'));
      | if latency < 1
      |     errordlg('Cannot have latency less than one.');
      |     set_param(gcb, 'latency', '1');
      | end
  sim_addr : hdlBasic/Gateway Out  inherit_from_input=off  bool_to_boolean=off  hdl_port=off  rows=1  columns=1  UseAsDAC=off  DACChannel='1'  interface=None  automatic_assignment=on  address_offset=hex2dec('00')  intf_name=''  intf_description=''  timing_constraint=None  locs_specified=off  LOCs={}  io_standard={}  XmcBlockStatus=1  maskContainerNames=group4  block_type=gatewayout  block_config=sysgen:gateway_out_config  block_width_w=590  block_height_w=620  block_width=620  block_height=750
  sim_data : hdlBasic/Gateway Out  inherit_from_input=off  bool_to_boolean=off  hdl_port=off  rows=1  columns=1  UseAsDAC=off  DACChannel='1'  interface=None  automatic_assignment=on  address_offset=hex2dec('00')  intf_name=''  intf_description=''  timing_constraint=None  locs_specified=off  LOCs={}  io_standard={}  XmcBlockStatus=1  maskContainerNames=group4  block_type=gatewayout  block_config=sysgen:gateway_out_config  block_width_w=590  block_height_w=620  block_width=620  block_height=750
  sim_we : hdlBasic/Gateway Out  inherit_from_input=off  bool_to_boolean=off  hdl_port=off  rows=1  columns=1  UseAsDAC=off  DACChannel='1'  interface=None  automatic_assignment=on  address_offset=hex2dec('00')  intf_name=''  intf_description=''  timing_constraint=None  locs_specified=off  LOCs={}  io_standard={}  XmcBlockStatus=1  maskContainerNames=group4  block_type=gatewayout  block_config=sysgen:gateway_out_config  block_width_w=590  block_height_w=620  block_width=620  block_height=750
  data_out : Outport  VectorParamsAs1DForOutWhenUnconnected=off
  wires:
  sfunc/1 -> data_out/1  "output"
  Data Type Conversion2/1 -> sfunc/3  "we"
  Data Type Conversion1/1 -> sfunc/2  "data_in"
  Data Type Conversion/1 -> sfunc/1  "addr"
  sim_we/1 -> Data Type Conversion2/1
  sim_data/1 -> Data Type Conversion1/1
  sim_addr/1 -> Data Type Conversion/1
  we/1 -> sim_we/1
  data/1 -> sim_data/1
  addr/1 -> sim_addr/1

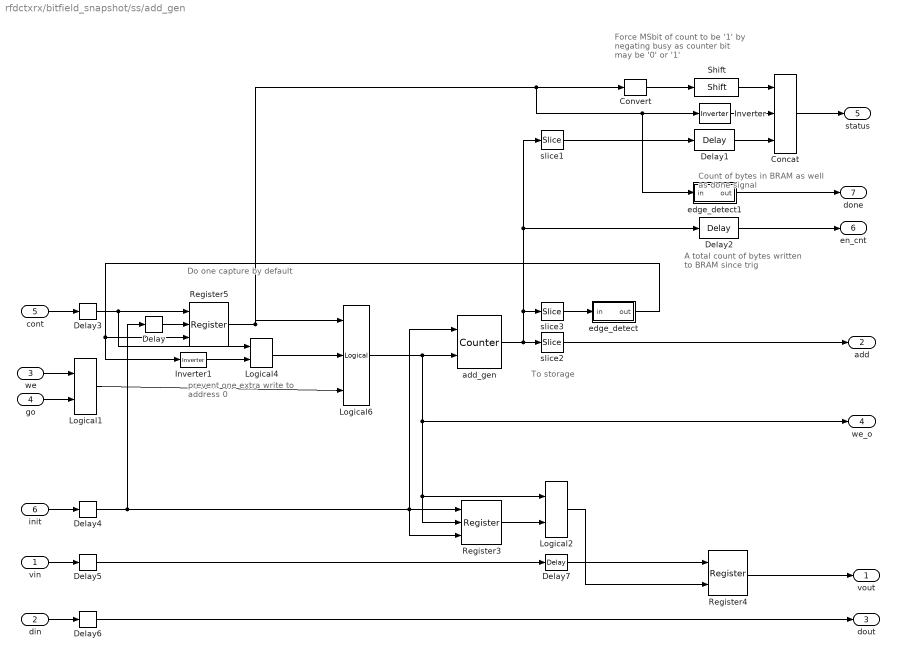
== system rfdctxrx/bitfield_snapshot/ss/add_gen ==
  note: Force MSbit of count
      | to be '1' by negating busy
      | as counter bit may be '0' or '1'
  note: A total count of
      | bytes written to
      | BRAM since trig
  note: Count of bytes in BRAM
      | as well as done signal
  note: Do one
      | capture by
      | default
  note: prevent one extra
      | write to address 0
  note: To storage
  vin : Inport
  din : Inport  Port=2
  we : Inport  Port=3
  go : Inport  Port=4
  cont : Inport  Port=5
  init : Inport  Port=6
  Concat : hdlBasic/Concat  num_inputs=3  XmcBlockStatus=1  maskContainerNames=group1  block_type=concat  block_config=sysgen:Concat_config
  Convert : hdlBasic/Convert  gui_display_data_type=Fixed-point  arith_type=Unsigned  n_bits=32-nsamples-log2(increment)-1  bin_pt=0  float_type=Single  exp_bits=8  fraction_bits=24  quantization=Truncate  overflow=Wrap  en=off  latency=0  pipeline=off  XmcBlockStatus=1  maskContainerNames=group2  block_type=convert  block_config=sysgen:Convert_config  block_width=595  block_height=885
  Delay{,3..6} (5 alike) : hdlBasic/Delay  rst=off  en=off  latency=1  reg_retiming=on  XmcBlockStatus=1  maskContainerNames=group1  block_type=delay  block_config=sysgen:Delay_config
  Delay1 : hdlBasic/Delay  rst=off  en=off  latency=1  reg_retiming=off  XmcBlockStatus=1  maskContainerNames=group1  block_type=delay  block_config=sysgen:Delay_config
  Delay2 : hdlBasic/Delay  rst=off  en=off  latency=1  reg_retiming=off  XmcBlockStatus=1  maskContainerNames=group1  block_type=delay  block_config=sysgen:Delay_config
  Delay7 : hdlBasic/Delay  rst=off  en=off  latency=1  reg_retiming=off  XmcBlockStatus=1  maskContainerNames=group1  block_type=delay  block_config=sysgen:Delay_config
  Inverter : hdlBasic/Inverter  en=off  latency=1  XmcBlockStatus=1  maskContainerNames=group2  block_type=inv  block_config=sysgen:Inverter_config
  Inverter1 : hdlBasic/Inverter  en=off  latency=0  XmcBlockStatus=1  maskContainerNames=group2  block_type=inv  block_config=sysgen:Inverter_config
  Logical1 : hdlBasic/Logical  logical_function=AND  inputs=2  en=off  latency=1  precision=Full  arith_type=Unsigned  n_bits=8  bin_pt=2  align_bp=on  overflow=[]  quantization=[]  XmcBlockStatus=1  maskContainerNames=tabcontainer1  block_type=logical  block_config=sysgen:Logical_config
  Logical2 : hdlBasic/Logical  logical_function=AND  inputs=2  en=off  latency=1  precision=Full  arith_type=Unsigned  n_bits=8  bin_pt=2  align_bp=on  overflow=[]  quantization=[]  XmcBlockStatus=1  maskContainerNames=tabcontainer1  block_type=logical  block_config=sysgen:Logical_config
  Logical4 : hdlBasic/Logical  logical_function=OR  inputs=2  en=off  latency=0  precision=Full  arith_type=Unsigned  n_bits=8  bin_pt=2  align_bp=on  overflow=[]  quantization=[]  XmcBlockStatus=1  maskContainerNames=tabcontainer1  block_type=logical  block_config=sysgen:Logical_config
  Logical6 : hdlBasic/Logical  logical_function=AND  inputs=3  en=off  latency=0  precision=Full  arith_type=Unsigned  n_bits=8  bin_pt=2  align_bp=on  overflow=[]  quantization=[]  XmcBlockStatus=1  maskContainerNames=tabcontainer1  block_type=logical  block_config=sysgen:Logical_config
  Register3 : hdlBasic/Register  init=0  rst=on  en=on  XmcBlockStatus=1  maskContainerNames=tabcontainer1  block_type=register  block_config=sysgen:Register_config
  Register4 : hdlBasic/Register  init=0  rst=off  en=on  XmcBlockStatus=1  maskContainerNames=tabcontainer1  block_type=register  block_config=sysgen:Register_config
  Register5 : hdlBasic/Register  init=1  rst=on  en=on  XmcBlockStatus=1  maskContainerNames=tabcontainer1  block_type=register  block_config=sysgen:Register_config
  Shift : hdlBasic/Shift  shift_dir=Left  shift_bits=32-nsamples-log2(increment)-1-1  en=off  latency=1  precision=Full  arith_type="Signed  (2's comp)"  n_bits=16  bin_pt=14  quantization=Truncate  overflow=Wrap  XmcBlockStatus=1  maskContainerNames=group2  block_type=shift  block_config=sysgen:Shift_config
  add_gen : hdlBasic/Counter  cnt_type=Free running  cnt_to=1  operation=Up  start_count=0  cnt_by_val=increment  arith_type=Unsigned  n_bits=counter_size  bin_pt=0  load_pin=off  rst=on  en=on  explicit_period=Explicit  period=1  use_behavioral_HDL=off  implementation=DSP48  use_rpm=on  XmcBlockStatus=1  maskContainerNames=group1  block_type=counter  block_config=sysgen:Counter_config  block_width=531  block_height=1023
  edge_detect : Subsystem  AncestorBlock=casper_library_misc/edge_detect  mask(edge_detect){edge=Both, polarity=Active High, x_in=[0 0.08 0.08 0.16 0.16 0.24 0.24 0.32 0.32 0.4], y_in=[-1 -1  1  1  1  1 -1 -1 -1 -1], x_out=[0.6 0.68 0.68 0.76 0.76 0.84 0.84 0.92 0.92 1], y_out=[-1 -1  1  1 -1 -1  1  1 -1 -1]}
      mask prompts: edge "Edge Type"; polarity "Output Polarity"; x_in "Input X Positions"; y_in "Input Y Positions"; x_out "Output X Positions"; y_out "Output Y Positions"
      mask help: Output is active for one-cycle after each edge of the specified type (i.e. rising, falling or both).
      mask init:
      | edge_detect_init(gcb,...
      |     'edge',edge,...
      |     'polarity',polarity,...
      |     'x_in',x_in,...
      |     'x_out',x_out,...
      |     'y_in',y_in,...
      |     'y_out',y_out);
      | 
      | x_in_num=str2num(getfield(getfield(get_param(gcb,'UserData'),'parameters'),'x_in'));
      | x_out_num=str2num(getfield(getfield(get_param(gcb,'UserData'),'parameters'),'x_out'));
      | y_in_num=str2num(getfield(getfield(get_param(gcb,'UserData'),'parameters'),'y_in'));
      | y_out_num=str2num(getfield(getfield(get_param(gcb,'UserData'),'parameters'),'y_out'));
      settings: AttributesFormatString=|
      | both edges
      | active high
      mask Help: Output is active for one-cycle after each edge of the specified type (i.e. rising, falling, or both).  Latency is zero.
      mask TypeOptions edge: Rising | Falling | Both
      mask TypeOptions polarity: Active High | Active Low
      mask Display:
      | plot(x_in_num,0.5+y_in_num*0.2);
      | plot(x_out_num,0.5+y_out_num*0.2);
  edge_detect1 : Subsystem  AncestorBlock=casper_library_scopes/snapshot/add_gen/edge_detect  mask(edge_detect){edge=Both, polarity=Active High, x_in=[0 0.08 0.08 0.16 0.16 0.24 0.24 0.32 0.32 0.4], y_in=[-1 -1  1  1  1  1 -1 -1 -1 -1], x_out=[0.6 0.68 0.68 0.76 0.76 0.84 0.84 0.92 0.92 1], y_out=[-1 -1  1  1 -1 -1  1  1 -1 -1]}
      mask prompts: edge "Edge Type"; polarity "Output Polarity"; x_in "Input X Positions"; y_in "Input Y Positions"; x_out "Output X Positions"; y_out "Output Y Positions"
      mask help: Output is active for one-cycle after each edge of the specified type (i.e. rising, falling or both).
      mask init: same as rfdctxrx/bitfield_snapshot/ss/add_gen/edge_detect
      settings: AttributesFormatString=|
      | both edges
      | active high
      mask Help: Output is active for one-cycle after each edge of the specified type (i.e. rising, falling, or both).  Latency is zero.
      mask TypeOptions edge: Rising | Falling | Both
      mask TypeOptions polarity: Active High | Active Low
      mask Display:
      | plot(x_in_num,0.5+y_in_num*0.2);
      | plot(x_out_num,0.5+y_out_num*0.2);
  slice1 : hdlBasic/Slice  nbits=nsamples+log2(increment)  boolean_output=off  mode=Lower Bit Location + Width  bit1=0  base1=LSB of Input  bit0=0  base0=LSB of Input  XmcBlockStatus=1  maskContainerNames=group1  block_type=slice  block_config=sysgen:Slice_config
  slice2 : hdlBasic/Slice  nbits=nsamples-burst_size  boolean_output=off  mode=Lower Bit Location + Width  bit1=0  base1=LSB of Input  bit0=log2(increment)+burst_size  base0=LSB of Input  XmcBlockStatus=1  maskContainerNames=group1  block_type=slice  block_config=sysgen:Slice_config
  slice3 : hdlBasic/Slice  nbits=1  boolean_output=on  mode=Lower Bit Location + Width  bit1=0  base1=MSB of Input  bit0=nsamples + log2(increment)  base0=LSB of Input  XmcBlockStatus=1  maskContainerNames=group1  block_type=slice  block_config=sysgen:Slice_config
  vout : Outport  VectorParamsAs1DForOutWhenUnconnected=off
  add : Outport  Port=2  VectorParamsAs1DForOutWhenUnconnected=off
  dout : Outport  Port=3  VectorParamsAs1DForOutWhenUnconnected=off
  we_o : Outport  Port=4  VectorParamsAs1DForOutWhenUnconnected=off
  status : Outport  Port=5  VectorParamsAs1DForOutWhenUnconnected=off
  en_cnt : Outport  Port=6  VectorParamsAs1DForOutWhenUnconnected=off
  done : Outport  Port=7  VectorParamsAs1DForOutWhenUnconnected=off
  wires:
  Delay6/1 -> dout/1
  Delay5/1 -> Delay7/1
  Delay4/1 -> Delay/1, Register3/1, Register3/3, add_gen/1
  Delay3/1 -> Register5/1, Logical4/1
  Delay7/1 -> Register4/1
  Logical1/1 -> Logical6/3
  go/1 -> Logical1/2
  we/1 -> Logical1/1
  Logical4/1 -> Logical6/2
  Inverter/1 -> Concat/2
  slice1/1 -> Delay1/1
  Delay1/1 -> Concat/3
  din/1 -> Delay6/1
  Delay2/1 -> en_cnt/1
  slice2/1 -> add/1
  Convert/1 -> Shift/1
  Concat/1 -> status/1
  Logical6/1 -> add_gen/2, Register3/2, Logical2/1, we_o/1
  init/1 -> Delay4/1
  slice3/1 -> edge_detect/1(in)
  Register5/1 -> Logical6/1, edge_detect1/1(in), Inverter/1, Convert/1
  add_gen/1 -> slice3/1, Delay2/1, slice1/1, slice2/1
  vin/1 -> Delay5/1
  Register3/1 -> Logical2/2
  Logical2/1 -> Register4/2
  Register4/1 -> vout/1
  edge_detect/1(out) -> Register5/3, Inverter1/1
  cont/1 -> Delay3/1
  Inverter1/1 -> Logical4/2
  Delay/1 -> Register5/2
  Shift/1 -> Concat/1
  edge_detect1/1(out) -> done/1

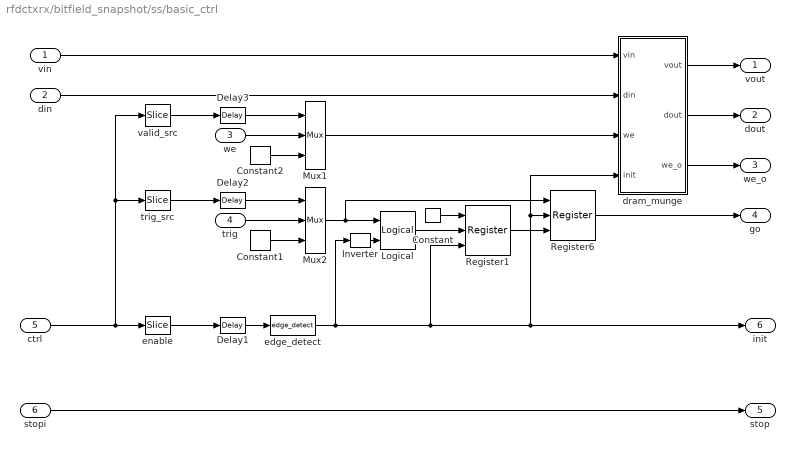
== system rfdctxrx/bitfield_snapshot/ss/basic_ctrl ==
  vin : Inport
  din : Inport  Port=2
  we : Inport  Port=3
  trig : Inport  Port=4
  ctrl : Inport  Port=5
  stopi : Inport  Port=6
  Constant : hdlBasic/Constant  const=1  gui_display_data_type=Boolean  arith_type=Boolean  n_bits=16  bin_pt=14  preci_type=Single  exp_width=8  frac_width=24  explicit_period=on  period=1  XmcBlockStatus=1  maskContainerNames=tabcontainer1  block_type=constant  block_config=sysgen:Constant_config
  Constant1 : hdlBasic/Constant  const=1  gui_display_data_type=Boolean  arith_type=Boolean  n_bits=1  bin_pt=0  preci_type=Single  exp_width=8  frac_width=24  explicit_period=on  period=1  XmcBlockStatus=1  maskContainerNames=tabcontainer1  block_type=constant  block_config=sysgen:Constant_config
  Constant2 : hdlBasic/Constant  const=1  gui_display_data_type=Boolean  arith_type=Boolean  n_bits=1  bin_pt=0  preci_type=Single  exp_width=8  frac_width=24  explicit_period=on  period=1  XmcBlockStatus=1  maskContainerNames=tabcontainer1  block_type=constant  block_config=sysgen:Constant_config
  Delay1 : hdlBasic/Delay  rst=off  en=off  latency=1  reg_retiming=off  XmcBlockStatus=1  maskContainerNames=group1  block_type=delay  block_config=sysgen:Delay_config
  Delay2 : hdlBasic/Delay  rst=off  en=off  latency=1  reg_retiming=off  XmcBlockStatus=1  maskContainerNames=group1  block_type=delay  block_config=sysgen:Delay_config
  Delay3 : hdlBasic/Delay  rst=off  en=off  latency=1  reg_retiming=off  XmcBlockStatus=1  maskContainerNames=group1  block_type=delay  block_config=sysgen:Delay_config
  Inverter : hdlBasic/Inverter  en=off  latency=0  XmcBlockStatus=1  maskContainerNames=group2  block_type=inv  block_config=sysgen:Inverter_config
  Logical : hdlBasic/Logical  logical_function=AND  inputs=2  en=off  latency=0  precision=Full  arith_type=Unsigned  n_bits=16  bin_pt=0  align_bp=on  overflow=[]  quantization=[]  XmcBlockStatus=1  maskContainerNames=tabcontainer1  block_type=logical  block_config=sysgen:Logical_config
  Mux1 : hdlBasic/Mux  inputs=2  en=off  latency=0  precision=Full  arith_type="Signed  (2's comp)"  n_bits=8  bin_pt=2  quantization=Truncate  overflow=Wrap  XmcBlockStatus=1  maskContainerNames=tabcontainer1  block_type=mux  block_config=sysgen:Mux_config
  Mux2 : hdlBasic/Mux  inputs=2  en=off  latency=0  precision=Full  arith_type="Signed  (2's comp)"  n_bits=8  bin_pt=2  quantization=Truncate  overflow=Wrap  XmcBlockStatus=1  maskContainerNames=tabcontainer1  block_type=mux  block_config=sysgen:Mux_config
  Register1 : hdlBasic/Register  init=0  rst=on  en=on  XmcBlockStatus=1  maskContainerNames=tabcontainer1  block_type=register  block_config=sysgen:Register_config
  Register6 : hdlBasic/Register  init=0  rst=on  en=on  XmcBlockStatus=1  maskContainerNames=tabcontainer1  block_type=register  block_config=sysgen:Register_config
  dram_munge : Subsystem  mask{dram=off, data_width=data_width}
      mask prompts: data_width "data width"
      mask init:
      | set_param(gcb,'LinkStatus','inactive');
      | if strcmp(dram,'on'),
      |     set_param([gcb,'/dram'], 'const', '1');
      | else,
      |     set_param([gcb,'/dram'], 'const', '0');
      | end
      | set_param([gcb,'/data_choice'], ...
      |         'precision', 'User Defined', ...
      |         'arith_type', 'Unsigned', ...
      |         'n_bits', num2str(data_width), 'bin_pt', '0', ...
      |         'quantization', 'Truncate', ...
      |         'overflow', 'Wrap');
  edge_detect : casper_library_misc/edge_detect  edge=Rising  polarity=Active High  x_in=[0 0.08 0.08 0.16 0.16 0.24 0.24 0.32 0.32 0.4]  y_in="[-1 -1  1  1  1  1  1  1  1  1]"  x_out=[0.6 0.68 0.68 0.76 0.76 0.84 0.84 0.92 0.92 1]  y_out="[-1 -1  1  1 -1 -1 -1 -1 -1 -1]"
      settings: SourceProductName=Misc
  enable : hdlBasic/Slice  nbits=1  boolean_output=on  mode=Lower Bit Location + Width  bit1=0  base1=LSB of Input  bit0=0  base0=LSB of Input  XmcBlockStatus=1  maskContainerNames=group1  block_type=slice  block_config=sysgen:Slice_config
  trig_src : hdlBasic/Slice  nbits=1  boolean_output=on  mode=Lower Bit Location + Width  bit1=0  base1=LSB of Input  bit0=1  base0=LSB of Input  XmcBlockStatus=1  maskContainerNames=group1  block_type=slice  block_config=sysgen:Slice_config
  valid_src : hdlBasic/Slice  nbits=1  boolean_output=on  mode=Lower Bit Location + Width  bit1=0  base1=LSB of Input  bit0=2  base0=LSB of Input  XmcBlockStatus=1  maskContainerNames=group1  block_type=slice  block_config=sysgen:Slice_config
  vout : Outport  VectorParamsAs1DForOutWhenUnconnected=off
  dout : Outport  Port=2  VectorParamsAs1DForOutWhenUnconnected=off
  we_o : Outport  Port=3  VectorParamsAs1DForOutWhenUnconnected=off
  go : Outport  Port=4  VectorParamsAs1DForOutWhenUnconnected=off
  stop : Outport  Port=5  VectorParamsAs1DForOutWhenUnconnected=off
  init : Outport  Port=6  VectorParamsAs1DForOutWhenUnconnected=off
  wires:
  Delay1/1 -> edge_detect/1
  Delay3/1 -> Mux1/1
  Delay2/1 -> Mux2/1
  dram_munge/1(vout) -> vout/1
  vin/1 -> dram_munge/1(vin)
  dram_munge/3(we_o) -> we_o/1
  dram_munge/2(dout) -> dout/1
  din/1 -> dram_munge/2(din)
  Inverter/1 -> Logical/2
  Mux2/1 -> Logical/1, Register6/1
  Register6/1 -> go/1
  trig/1 -> Mux2/2
  Mux1/1 -> dram_munge/3(we)
  we/1 -> Mux1/2
  ctrl/1 -> enable/1, valid_src/1, trig_src/1
  edge_detect/1 -> Inverter/1, Register1/3, dram_munge/4(init), Register6/2, init/1
  enable/1 -> Delay1/1
  Constant1/1 -> Mux2/3
  Constant2/1 -> Mux1/3
  trig_src/1 -> Delay2/1
  valid_src/1 -> Delay3/1
  Constant/1 -> Register1/1
  Register1/1 -> Register6/3
  Logical/1 -> Register1/2
  stopi/1 -> stop/1
